simulink model "Sim2Real_whole_body_motion"  (R2025a)
settings: Solver=FixedStepDiscrete  StartTime=0.0  StopTime=19  FixedStep=Ts_1ms  MaxStep=0.002  RelTol=1e-3
InitFcn:
  | modelFile = get_param(bdroot,'FileName');
  | if isempty(modelFile)
  |     error('The model must be saved before running InitFcn.');
  | end
  | 
  | % Folder where the .slx model is located
  | modelFolder = fileparts(char(modelFile));
  | 
  | % Find the parent folder named "resources" by going upwards
  | currentFolder  = modelFolder;
  | materialFolder = '';
  | 
  | while true
  |     [parentFolder, currentName] = fileparts(currentFolder);
  | 
  |     if strcmpi(currentName, 'resources')
  |         materialFolder = currentFolder;
  |         break;
  |     end
  | 
  |     if strcmp(parentFolder, currentFolder)
  |         error('Could not find a parent folder named "resources" starting from: %s', modelFolder);
  |     end
  | 
  |     currentFolder = parentFolder;
  | end
  | 
  | % Search recursively for the MuJoCo XML inside "material"
  | xmlSearch = dir(fullfile(materialFolder, '**', 'unitree_G1.xml'));
  | 
  | if isempty(xmlSearch)
  |     error('MuJoCo XML file not found inside material folder: %s', materialFolder);
  | elseif numel(xmlSearch) > 1
  |     error('Multiple unitree_G1.xml files found inside material folder. Leave only one valid XML.');
  | end
  | 
  | mujocoFolder = xmlSearch(1).folder;
  | xmlFullPath  = fullfile(xmlSearch(1).folder, xmlSearch(1).name);
  | 
  | % Save in base workspace in case you want to inspect them
  | assignin('base','modelFolder',modelFolder);
  | assignin('base','materialFolder',materialFolder);
  | assignin('base','mujocoFolder',mujocoFolder);
  | assignin('base','xmlFullPath',xmlFullPath);
  | 
  | % Final existence check
  | if exist(xmlFullPath,'file') ~= 2
  |     error('MuJoCo XML file not found: %s', xmlFullPath);
  | end
  | 
  | % Add the XML folder to the path so WHICH can find it
  | addpath(mujocoFolder, '-begin');
  | rehash path;
  | 
  | % Run launcher from the same folder as the model
  | launcherFile = fullfile(modelFolder, 'launcher_whole_body_motion.mlx');
  | if exist(launcherFile,'file') == 2
  |     run(launcherFile);
  | else
  |     error('Launcher file not found: %s', launcherFile);
  | ... (+17 lines)
StopFcn:
  | drawnow; pause(0.05);
  | 
  | % Stop figures
  | tags = {'G1_IMUState','G1_MotorState'};
  | for k = 1:numel(tags)
  |     delete(findall(0,'Type','uifigure','Tag',tags{k}));
  |     delete(findall(0,'Type','figure' , 'Tag',tags{k}));
  | end
  | 
  | 
  | % Whole-body CSV export
  | addpath(fileparts(get_param('Sim2Real_whole_body_motion','FileName')));
  | whole_body_motion_csv('save');
undefined symbols (not defined in the file or in its folder): crc, mode_machine, mode_pr, motor_cmd, reserve, Ts_1ms, Ts_2ms
libraries: ros2lib x3, mjLib x1
(part 3 of 3)

== matlab function Sim2Real_whole_body_motion/SIM2REAL VARIANT SUBSYSTEM/MuJoCo SUBSYSTEM/MuJoCo SUBSYSTEM/JOINT COMMAND/CRANE ==
  data: start_enable input; crane_tau output; ankle_pitch_tau output; grip_open output; P_MACHINE_DATA parameter
function [crane_tau, ankle_pitch_tau, grip_open] = crane_function(start_enable, P_MACHINE_DATA)

Ts      = P_MACHINE_DATA.Ts_1ms;  
u_hold  = 1250;
u_low   = 440; % before 440
u_high  = 730; % before 730
t_wait  = 0.1; % before 1.7
t_kick  = 0.9;
t_ramp  = 2.5;
t_raise = 1.7;
t_pre   = 0.5;
grip_base     = -0.08;      % max value -0.15
grip_hold     =  1.2;       % max value 2.45
grip_wait_SE1 = 10.0;
crane_boost_tau   = 780;   % 800 to go up, 720 to hold
crane_boost_delay = 0.05;  
crane_boost_time  = 2.0;   

persistent t_elapsed grip_latched se1_steps boost_stage boost_steps

if isempty(t_elapsed)
    t_elapsed    = 0;
    grip_latched = false;
    se1_steps    = uint32(0);
    boost_stage  = uint8(0);
    boost_steps  = uint32(0);
end

if start_enable == 0
    crane_tau       = u_hold;
    ankle_pitch_tau = 0.3;
    grip_open       = grip_base;
    t_elapsed    = 0;
    grip_latched = false;
    se1_steps    = uint32(0);
    boost_stage  = uint8(0);
    boost_steps  = uint32(0);
    return;
end

t1 = t_wait;
t2 = t_wait + t_kick;

if t_elapsed < t1
    ankle_pitch_tau = 0;
elseif t_elapsed < t2
    ankle_pitch_tau = -0.35;
else
    ankle_pitch_tau = 0;
end

if t_elapsed < t_ramp
    alphaA = t_elapsed / t_ramp;   
    if alphaA < 0, alphaA = 0; end
    if alphaA > 1, alphaA = 1; end
    crane_tau = u_hold + (u_low - u_hold) * alphaA;
else
    crane_tau = u_low;
end

t_raise_start = 2.1;

if t_elapsed >= t_raise_start
    tauB = t_elapsed - t_raise_start;
    if tauB < t_raise
        alphaB = tauB / t_raise;
        if alphaB < 0, alphaB = 0; end
        if alphaB > 1, alphaB = 1; end
        crane_tau = u_low + (u_high - u_low) * alphaB;
    else
        crane_tau = u_high;
    end
end

se1_steps = se1_steps + uint32(1);

if ~grip_latched
    if double(se1_steps) * Ts >= grip_wait_SE1
        grip_latched = true;
        boost_stage = uint8(1); 
        boost_steps = uint32(0);
    end
end

if grip_latched
    grip_open = grip_hold;  
else
    grip_open = grip_base; 
end

if boost_stage ~= uint8(0)
    boost_steps = boost_steps + uint32(1);
    t_boost = double(boost_steps) * Ts;
    if boost_stage == uint8(1)
        % delay stage
        if t_boost >= crane_boost_delay
            boost_stage = uint8(2);
            boost_steps = uint32(0); 
        end
    elseif boost_stage == uint8(2)
        if (double(boost_steps) * Ts) <= crane_boost_time
            crane_tau = crane_boost_tau;
        else
            boost_stage = uint8(0);    
        end
    end
end

t_elapsed = t_elapsed + Ts;
end
